simulink model "P2_C"  (R2024b)
settings: Solver=VariableStepAuto  StartTime=0.0  StopTime=100  RelTol=1e-3
settings Model: Creator=sepeh  LastModifiedBy=sepeh

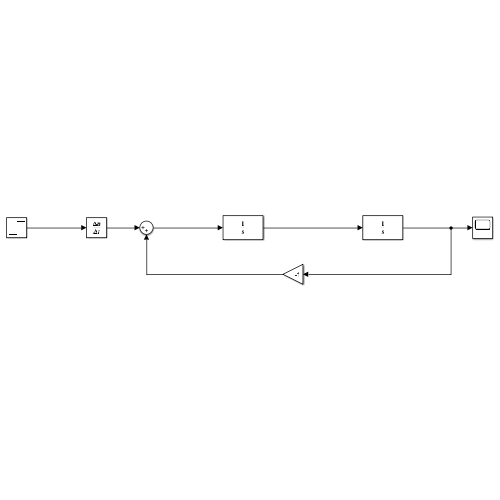
[thumbnail: Simulink's stored preview of the top-level diagram]
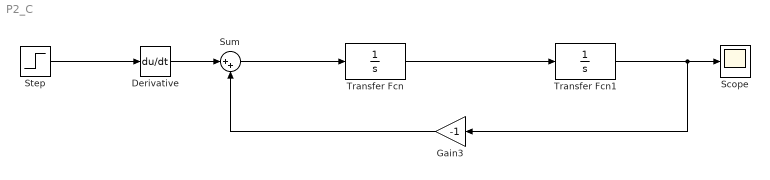
== system P2_C ==
  Derivative : Derivative
  Gain3 : Gain  Gain=-1
  Scope : Scope
  Step : Step  SampleTime=0
  Sum : Sum  Inputs=|++
  Transfer Fcn : TransferFcn  Denominator="[1  0]"
  Transfer Fcn1 : TransferFcn  Denominator="[1  0]"
  wires:
  Step/1 -> Derivative/1
  Derivative/1 -> Sum/1
  Gain3/1 -> Sum/2
  Sum/1 -> Transfer Fcn/1
  Transfer Fcn/1 -> Transfer Fcn1/1
  Transfer Fcn1/1 -> Gain3/1, Scope/1
